simulink model "simrt_serial_com56"  (R2024b)
settings: Solver=FixedStepDiscrete  StartTime=0.0  StopTime=inf  FixedStep=0.001  RelTol=1e-3
model workspace (MAT data in the model file):
  Serial_Enable = Simulink.Parameter
  Serial_Enable.Value = 0
  Serial_Enable.Complexity = 'real'
  Serial_Enable.Dimensions = [1 1]
  Serial_Enable.Description = '0 stops transmission and clears bench counters; 1 starts alternating COM5/COM6 frames.'
  Serial_Enable.DataType = 'uint8'
  Serial_Enable.Min = 0
  Serial_Enable.Max = 1
libraries: simrt_serial_library x6
settings Model: Creator=yonggang.zhang  LastModifiedBy=yonggang.zhang
settings OptimizationCC: EnhancedBackFolding=on  PassReuseOutputArgsAs=Individual arguments  ZeroExternalMemoryAtStartup=off  ZeroInternalMemoryAtStartup=off  MaxStackSize=64  OptimizeBlockOrder=speed  DifferentSizesBufferReuse=on  OptimizationCustomize=off  EfficientTunableParamExpr=on
settings DebuggingCC: ParameterTunabilityLossMsg=error
settings HardwareCC: ProdBitPerLong=64  ProdHWDeviceType=Intel->x86-64 (Linux 64)
settings SFSimCC: MATLABDynamicMemAlloc=off
settings RTWCC: Description=Embedded Coder  SystemTargetFile=ert.tlc  HardwareBoard=SimRT  TLCOptions="-aInlineSetEventsForThisBaseRateFcn=TLC_FALSE -aSuppressMultiTaskScheduler=TLC_FALSE  -aRateBasedStepFcn=0"  TemplateMakefile=ert_default_tmf  Toolchain=SimRT portable-linux-toolchain
settings CodeAppCC: ForceParamTrailComments=on  IgnoreCustomStorageClasses=off  OperatorAnnotations=on  SimulinkDataObjDesc=on  SFDataObjDesc=on  InsertBlockDesc=on
settings ERTTargetCC: ExtMode=on  ExtModeTransport=2  ExtModeStaticAlloc=on  ExtModeMexFile=ext_xcp  ExtModeIntrfLevel=Level2 - Open  InlinedParameterPlacement=Hierarchical

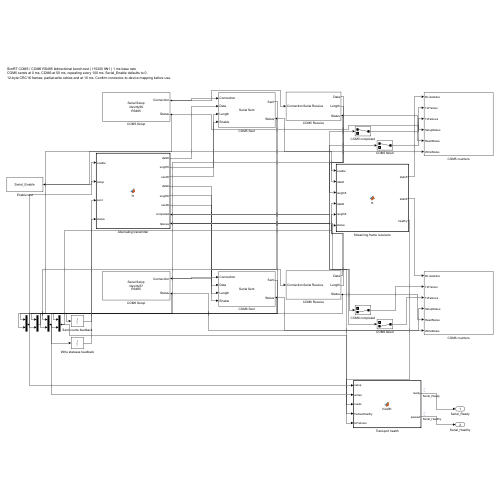
[thumbnail: Simulink's stored preview of the top-level diagram]
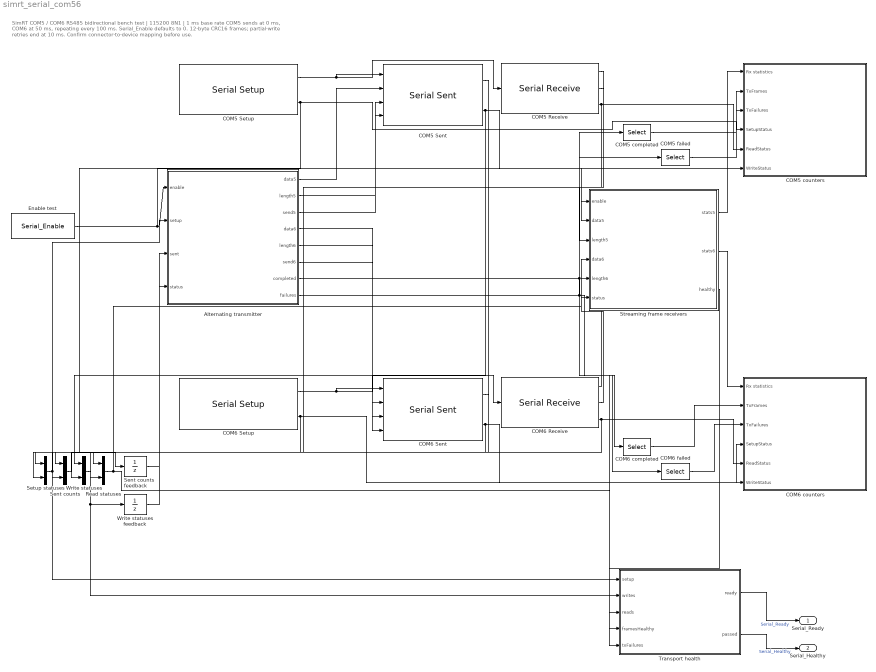
== system simrt_serial_com56 ==
  note: SimRT COM5 / COM6 RS485 bidirectional bench test | 115200 8N1 | 1 ms base rate
      | COM5 sends at 0 ms, COM6 at 50 ms, repeating every 100 ms. Serial_Enable defaults to 0.
      | 12-byte CRC16 frames; partial-write retries end at 10 ms. Confirm connector-to-device mapping before use.
  Alternating transmitter : MATLAB Function  TreatAsAtomicUnit=on
  COM5 Receive : simrt_serial_library/Serial Receive  BufferSize=64
  COM5 Sent : simrt_serial_library/Serial Sent
  COM5 Setup : simrt_serial_library/Serial Setup  Device=/dev/ttyS6  BaudRate=115200  DataBits=8  Parity=None  StopBits=1  Mode=RS485  RS485Direction=Hardware auto  RTSOnSend=true  DelayBeforeSendMs=0  DelayAfterSendMs=0  SampleTime=0.001
  COM5 completed : Selector  InputPortWidth=2  IndexOptions=Index vector (dialog)  Indices=1  OutputSizes=1
  COM5 counters : Subsystem
  COM5 failed : Selector  InputPortWidth=2  IndexOptions=Index vector (dialog)  Indices=1  OutputSizes=1
  COM6 Receive : simrt_serial_library/Serial Receive  BufferSize=64
  COM6 Sent : simrt_serial_library/Serial Sent
  COM6 Setup : simrt_serial_library/Serial Setup  Device=/dev/ttyS7  BaudRate=115200  DataBits=8  Parity=None  StopBits=1  Mode=RS485  RS485Direction=Hardware auto  RTSOnSend=true  DelayBeforeSendMs=0  DelayAfterSendMs=0  SampleTime=0.001
  COM6 completed : Selector  InputPortWidth=2  IndexOptions=Index vector (dialog)  Indices=2  OutputSizes=1
  COM6 counters : Subsystem
  COM6 failed : Selector  InputPortWidth=2  IndexOptions=Index vector (dialog)  Indices=2  OutputSizes=1
  Enable test : Constant  Value=Serial_Enable  SampleTime=0.001
  Read statuses : Mux  Inputs=2
  Sent counts : Mux  Inputs=2
  Sent counts feedback : UnitDelay  InitialCondition=uint32(0)  SampleTime=0.001  HasFrameUpgradeWarning=on
  Setup statuses : Mux  Inputs=2
  Streaming frame receivers : MATLAB Function  TreatAsAtomicUnit=on
  Transport health : MATLAB Function  TreatAsAtomicUnit=on
  Write statuses : Mux  Inputs=2
  Write statuses feedback : UnitDelay  InitialCondition=int32(0)  SampleTime=0.001  HasFrameUpgradeWarning=on
  Serial_Ready : Outport
  Serial_Healthy : Outport  Port=2
  wires:
  COM5 Setup/1 -> COM5 Sent/1, COM5 Receive/1
  Alternating transmitter/1(data5) -> COM5 Sent/2
  Alternating transmitter/2(length5) -> COM5 Sent/3
  Alternating transmitter/3(send5) -> COM5 Sent/4
  COM5 Receive/1 -> Streaming frame receivers/2(data5)
  COM5 Receive/2 -> Streaming frame receivers/3(length5)
  Streaming frame receivers/1(stats5) -> COM5 counters/1(Rx statistics)
  Alternating transmitter/7(completed) -> COM5 completed/1, COM6 completed/1
  Alternating transmitter/8(failures) -> COM5 failed/1, COM6 failed/1, Transport health/5(txFailures)
  COM5 completed/1 -> COM5 counters/2(TxFrames)
  COM5 failed/1 -> COM5 counters/3(TxFailures)
  COM5 Setup/2 -> COM5 counters/4(SetupStatus), Setup statuses/1
  COM5 Receive/3 -> COM5 counters/5(ReadStatus), Read statuses/1
  COM5 Sent/2 -> COM5 counters/6(WriteStatus), Write statuses/1
  COM6 Setup/1 -> COM6 Sent/1, COM6 Receive/1
  Alternating transmitter/4(data6) -> COM6 Sent/2
  Alternating transmitter/5(length6) -> COM6 Sent/3
  Alternating transmitter/6(send6) -> COM6 Sent/4
  COM6 Receive/1 -> Streaming frame receivers/4(data6)
  COM6 Receive/2 -> Streaming frame receivers/5(length6)
  Streaming frame receivers/2(stats6) -> COM6 counters/1(Rx statistics)
  COM6 completed/1 -> COM6 counters/2(TxFrames)
  COM6 failed/1 -> COM6 counters/3(TxFailures)
  COM6 Setup/2 -> COM6 counters/4(SetupStatus), Setup statuses/2
  COM6 Receive/3 -> COM6 counters/5(ReadStatus), Read statuses/2
  COM6 Sent/2 -> COM6 counters/6(WriteStatus), Write statuses/2
  COM5 Sent/1 -> Sent counts/1
  COM6 Sent/1 -> Sent counts/2
  Sent counts/1 -> Sent counts feedback/1
  Write statuses/1 -> Write statuses feedback/1, Transport health/2(writes)
  Enable test/1 -> Alternating transmitter/1(enable), Streaming frame receivers/1(enable)
  Setup statuses/1 -> Alternating transmitter/2(setup), Transport health/1(setup)
  Sent counts feedback/1 -> Alternating transmitter/3(sent)
  Write statuses feedback/1 -> Alternating transmitter/4(status)
  Read statuses/1 -> Streaming frame receivers/6(status), Transport health/3(reads)
  Streaming frame receivers/3(healthy) -> Transport health/4(framesHealthy)
  Transport health/1(ready) -> Serial_Ready/1  "Serial_Ready"
  Transport health/2(passed) -> Serial_Healthy/1  "Serial_Healthy"

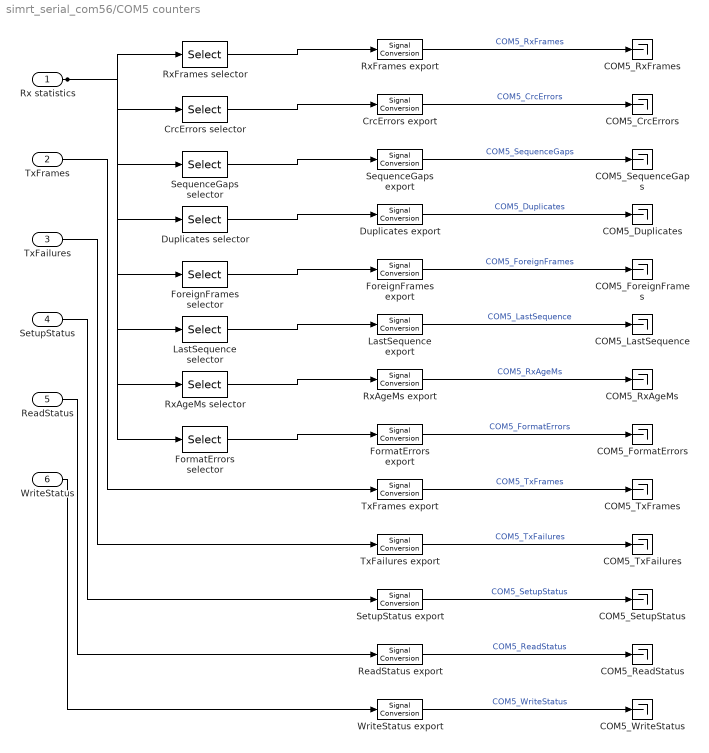
== system simrt_serial_com56/COM5 counters ==
  Rx statistics : Inport
  TxFrames : Inport  Port=2
  TxFailures : Inport  Port=3
  SetupStatus : Inport  Port=4
  ReadStatus : Inport  Port=5
  WriteStatus : Inport  Port=6
  COM5_CrcErrors : Terminator
  COM5_Duplicates : Terminator
  COM5_ForeignFrames : Terminator
  COM5_FormatErrors : Terminator
  COM5_LastSequence : Terminator
  COM5_ReadStatus : Terminator
  COM5_RxAgeMs : Terminator
  COM5_RxFrames : Terminator
  COM5_SequenceGaps : Terminator
  COM5_SetupStatus : Terminator
  COM5_TxFailures : Terminator
  COM5_TxFrames : Terminator
  COM5_WriteStatus : Terminator
  CrcErrors export : SignalConversion  OverrideOpt=off
  CrcErrors selector : Selector  InputPortWidth=8  IndexOptions=Index vector (dialog)  Indices=2  OutputSizes=1
  Duplicates export : SignalConversion  OverrideOpt=off
  Duplicates selector : Selector  InputPortWidth=8  IndexOptions=Index vector (dialog)  Indices=4  OutputSizes=1
  ForeignFrames export : SignalConversion  OverrideOpt=off
  ForeignFrames selector : Selector  InputPortWidth=8  IndexOptions=Index vector (dialog)  Indices=5  OutputSizes=1
  FormatErrors export : SignalConversion  OverrideOpt=off
  FormatErrors selector : Selector  InputPortWidth=8  IndexOptions=Index vector (dialog)  Indices=8  OutputSizes=1
  LastSequence export : SignalConversion  OverrideOpt=off
  LastSequence selector : Selector  InputPortWidth=8  IndexOptions=Index vector (dialog)  Indices=6  OutputSizes=1
  ReadStatus export : SignalConversion  OverrideOpt=off
  RxAgeMs export : SignalConversion  OverrideOpt=off
  RxAgeMs selector : Selector  InputPortWidth=8  IndexOptions=Index vector (dialog)  Indices=7  OutputSizes=1
  RxFrames export : SignalConversion  OverrideOpt=off
  RxFrames selector : Selector  InputPortWidth=8  IndexOptions=Index vector (dialog)  Indices=1  OutputSizes=1
  SequenceGaps export : SignalConversion  OverrideOpt=off
  SequenceGaps selector : Selector  InputPortWidth=8  IndexOptions=Index vector (dialog)  Indices=3  OutputSizes=1
  SetupStatus export : SignalConversion  OverrideOpt=off
  TxFailures export : SignalConversion  OverrideOpt=off
  TxFrames export : SignalConversion  OverrideOpt=off
  WriteStatus export : SignalConversion  OverrideOpt=off
  wires:
  Rx statistics/1 -> RxFrames selector/1, CrcErrors selector/1, SequenceGaps selector/1, Duplicates selector/1, ForeignFrames selector/1, LastSequence selector/1, RxAgeMs selector/1, FormatErrors selector/1
  RxFrames selector/1 -> RxFrames export/1
  RxFrames export/1 -> COM5_RxFrames/1  "COM5_RxFrames"
  CrcErrors selector/1 -> CrcErrors export/1
  CrcErrors export/1 -> COM5_CrcErrors/1  "COM5_CrcErrors"
  SequenceGaps selector/1 -> SequenceGaps export/1
  SequenceGaps export/1 -> COM5_SequenceGaps/1  "COM5_SequenceGaps"
  Duplicates selector/1 -> Duplicates export/1
  Duplicates export/1 -> COM5_Duplicates/1  "COM5_Duplicates"
  ForeignFrames selector/1 -> ForeignFrames export/1
  ForeignFrames export/1 -> COM5_ForeignFrames/1  "COM5_ForeignFrames"
  LastSequence selector/1 -> LastSequence export/1
  LastSequence export/1 -> COM5_LastSequence/1  "COM5_LastSequence"
  RxAgeMs selector/1 -> RxAgeMs export/1
  RxAgeMs export/1 -> COM5_RxAgeMs/1  "COM5_RxAgeMs"
  FormatErrors selector/1 -> FormatErrors export/1
  FormatErrors export/1 -> COM5_FormatErrors/1  "COM5_FormatErrors"
  TxFrames/1 -> TxFrames export/1
  TxFrames export/1 -> COM5_TxFrames/1  "COM5_TxFrames"
  TxFailures/1 -> TxFailures export/1
  TxFailures export/1 -> COM5_TxFailures/1  "COM5_TxFailures"
  SetupStatus/1 -> SetupStatus export/1
  SetupStatus export/1 -> COM5_SetupStatus/1  "COM5_SetupStatus"
  ReadStatus/1 -> ReadStatus export/1
  ReadStatus export/1 -> COM5_ReadStatus/1  "COM5_ReadStatus"
  WriteStatus/1 -> WriteStatus export/1
  WriteStatus export/1 -> COM5_WriteStatus/1  "COM5_WriteStatus"

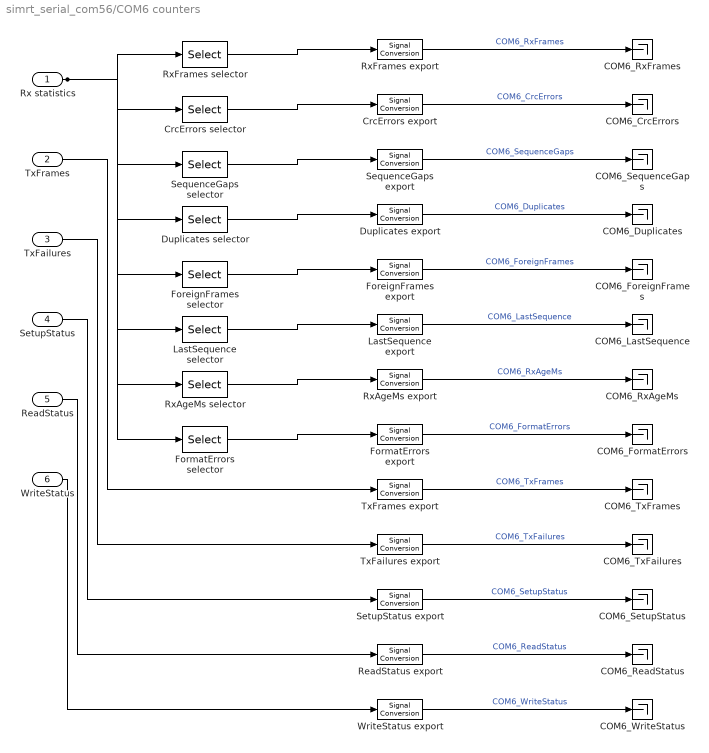
== system simrt_serial_com56/COM6 counters ==
  Rx statistics : Inport
  TxFrames : Inport  Port=2
  TxFailures : Inport  Port=3
  SetupStatus : Inport  Port=4
  ReadStatus : Inport  Port=5
  WriteStatus : Inport  Port=6
  COM6_CrcErrors : Terminator
  COM6_Duplicates : Terminator
  COM6_ForeignFrames : Terminator
  COM6_FormatErrors : Terminator
  COM6_LastSequence : Terminator
  COM6_ReadStatus : Terminator
  COM6_RxAgeMs : Terminator
  COM6_RxFrames : Terminator
  COM6_SequenceGaps : Terminator
  COM6_SetupStatus : Terminator
  COM6_TxFailures : Terminator
  COM6_TxFrames : Terminator
  COM6_WriteStatus : Terminator
  CrcErrors export : SignalConversion  OverrideOpt=off
  CrcErrors selector : Selector  InputPortWidth=8  IndexOptions=Index vector (dialog)  Indices=2  OutputSizes=1
  Duplicates export : SignalConversion  OverrideOpt=off
  Duplicates selector : Selector  InputPortWidth=8  IndexOptions=Index vector (dialog)  Indices=4  OutputSizes=1
  ForeignFrames export : SignalConversion  OverrideOpt=off
  ForeignFrames selector : Selector  InputPortWidth=8  IndexOptions=Index vector (dialog)  Indices=5  OutputSizes=1
  FormatErrors export : SignalConversion  OverrideOpt=off
  FormatErrors selector : Selector  InputPortWidth=8  IndexOptions=Index vector (dialog)  Indices=8  OutputSizes=1
  LastSequence export : SignalConversion  OverrideOpt=off
  LastSequence selector : Selector  InputPortWidth=8  IndexOptions=Index vector (dialog)  Indices=6  OutputSizes=1
  ReadStatus export : SignalConversion  OverrideOpt=off
  RxAgeMs export : SignalConversion  OverrideOpt=off
  RxAgeMs selector : Selector  InputPortWidth=8  IndexOptions=Index vector (dialog)  Indices=7  OutputSizes=1
  RxFrames export : SignalConversion  OverrideOpt=off
  RxFrames selector : Selector  InputPortWidth=8  IndexOptions=Index vector (dialog)  Indices=1  OutputSizes=1
  SequenceGaps export : SignalConversion  OverrideOpt=off
  SequenceGaps selector : Selector  InputPortWidth=8  IndexOptions=Index vector (dialog)  Indices=3  OutputSizes=1
  SetupStatus export : SignalConversion  OverrideOpt=off
  TxFailures export : SignalConversion  OverrideOpt=off
  TxFrames export : SignalConversion  OverrideOpt=off
  WriteStatus export : SignalConversion  OverrideOpt=off
  wires:
  Rx statistics/1 -> RxFrames selector/1, CrcErrors selector/1, SequenceGaps selector/1, Duplicates selector/1, ForeignFrames selector/1, LastSequence selector/1, RxAgeMs selector/1, FormatErrors selector/1
  RxFrames selector/1 -> RxFrames export/1
  RxFrames export/1 -> COM6_RxFrames/1  "COM6_RxFrames"
  CrcErrors selector/1 -> CrcErrors export/1
  CrcErrors export/1 -> COM6_CrcErrors/1  "COM6_CrcErrors"
  SequenceGaps selector/1 -> SequenceGaps export/1
  SequenceGaps export/1 -> COM6_SequenceGaps/1  "COM6_SequenceGaps"
  Duplicates selector/1 -> Duplicates export/1
  Duplicates export/1 -> COM6_Duplicates/1  "COM6_Duplicates"
  ForeignFrames selector/1 -> ForeignFrames export/1
  ForeignFrames export/1 -> COM6_ForeignFrames/1  "COM6_ForeignFrames"
  LastSequence selector/1 -> LastSequence export/1
  LastSequence export/1 -> COM6_LastSequence/1  "COM6_LastSequence"
  RxAgeMs selector/1 -> RxAgeMs export/1
  RxAgeMs export/1 -> COM6_RxAgeMs/1  "COM6_RxAgeMs"
  FormatErrors selector/1 -> FormatErrors export/1
  FormatErrors export/1 -> COM6_FormatErrors/1  "COM6_FormatErrors"
  TxFrames/1 -> TxFrames export/1
  TxFrames export/1 -> COM6_TxFrames/1  "COM6_TxFrames"
  TxFailures/1 -> TxFailures export/1
  TxFailures export/1 -> COM6_TxFailures/1  "COM6_TxFailures"
  SetupStatus/1 -> SetupStatus export/1
  SetupStatus export/1 -> COM6_SetupStatus/1  "COM6_SetupStatus"
  ReadStatus/1 -> ReadStatus export/1
  ReadStatus export/1 -> COM6_ReadStatus/1  "COM6_ReadStatus"
  WriteStatus/1 -> WriteStatus export/1
  WriteStatus export/1 -> COM6_WriteStatus/1  "COM6_WriteStatus"

== matlab function simrt_serial_com56/Streaming frame receivers ==
  data: enable input; stats5 output; data5 input; length5 input; data6 input; length6 input; status input; stats6 output; healthy output
function [stats5, stats6, healthy] = rx(enable, data5, length5, data6, length6, status)
[stats5, stats6, healthy] = simrtlinux.serial.duplexReceive(enable, data5, length5, data6, length6, status);
end

== matlab function simrt_serial_com56/Alternating transmitter ==
  data: enable input; data5 output; setup input; sent input; status input; length5 output; send5 output; data6 output; length6 output; send6 output; completed output; failures output
function [data5, length5, send5, data6, length6, send6, completed, failures] = tx(enable, setup, sent, status)
[data5, length5, send5, data6, length6, send6, completed, failures] = simrtlinux.serial.duplexTransmit(enable, setup, sent, status);
end

== matlab function simrt_serial_com56/Transport health ==
  data: setup input; ready output; writes input; reads input; framesHealthy input; txFailures input; passed output
function [ready, passed] = health(setup, writes, reads, framesHealthy, txFailures)
ready = all(setup == 0) && all(reads == 0) && all(writes == 0 | writes == -11);
passed = ready && framesHealthy && all(txFailures == 0);
end
